simulink library "fmPlaneAttiIndi_lib"  (R2018b)
settings: Solver=VariableStepAuto  StartTime=0.0  StopTime=10.0  RelTol=1e-3
undefined symbols (not defined in the file or in its folder): DiscIntNeverNeededParam, fm_atti
libraries: filters_lib x3, ca_lib x1, sensors_lib x1, $bdroot x1
settings Model: Creator=Ybeyer  LastModifiedBy=yannic
settings SFSimCC: SimUseLocalCustomCode=off
settings RTWCC: RTWUseLocalCustomCode=off
settings CodeAppCC: StateflowObjectComments=on

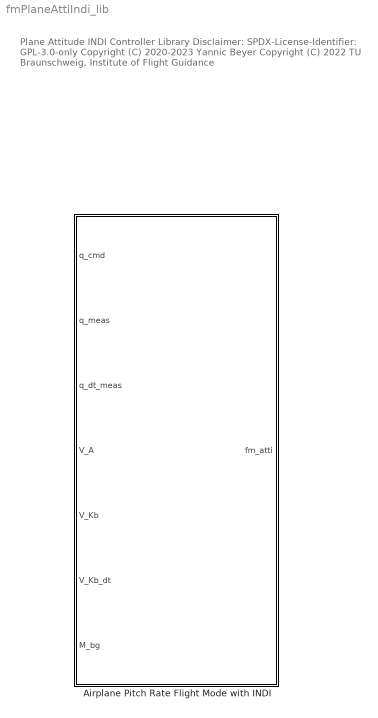
== system fmPlaneAttiIndi_lib ==
  note: Plane Attitude INDI Controller Library
      |
      | Disclaimer:
      | SPDX-License-Identifier: GPL-3.0-only
      |
      | Copyright (C) 2020-2023 Yannic Beyer
      | Copyright (C) 2022 TU Braunschweig, Institute of Flight Guidance
  Airplane Pitch Rate Flight Mode with INDI : Subsystem  mask{fm=fm_atti}
      mask prompts: fm "Multicopter Attitude Flight Mode (INDI) struct"
      mask DialogControl DescGroupVar Prompt: Multicopter Attitude Flight Mode with INDI and reduced attitude control
      mask DialogControl DescTextVar Prompt: Controller is basically implemented according to [1]
      mask DialogControl Control2 Prompt: [1] Sun, S., Baert, M., Van Schijndel, B. S., & De Visser, C. (2020, May). Upset Recovery Control for Quadrotors Subjected to a Complete Rotor Failure from Large Initial Disturbances. In 2020 IEEE International Conference on Robotics and Automation (ICRA) (pp. 4273-4279). IEEE.
      mask DialogControl Control3 Prompt: To initialize an attitude flight mode parameters struct see fmCopterAttiIndiLoadParams

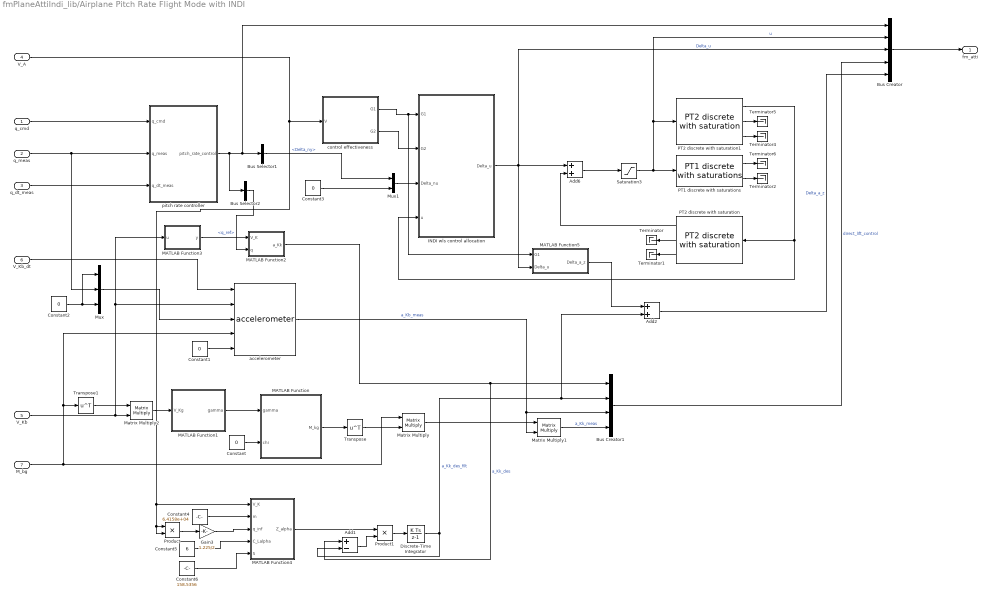
== system fmPlaneAttiIndi_lib/Airplane Pitch Rate Flight Mode with INDI ==
  q_cmd : Inport  SampleTime=fm.sample_time
  q_meas : Inport  Port=2  SampleTime=fm.sample_time
  q_dt_meas : Inport  Port=3  SampleTime=fm.sample_time
  V_A : Inport  Port=4  SampleTime=fm.sample_time
  V_Kb : Inport  Port=5  SampleTime=fm.sample_time
  V_Kb_dt : Inport  Port=6  SampleTime=fm.sample_time
  M_bg : Inport  Port=7  SampleTime=fm.sample_time
  Add1 : Sum  Inputs=+-
  Add2 : Sum
  Add6 : Sum
  Bus Creator : BusCreator  Inputs=5
  Bus Creator1 : BusCreator  Inputs=4
  Bus Selector1 : BusSelector  OutputSignals=pseudo_control.Delta_ny
  Bus Selector2 : BusSelector  OutputSignals=reference.q_ref
  Constant : Constant  Value=0
  Constant1 : Constant  Value=0  VectorParams1D=off
  Constant2 : Constant  Value=0
  Constant3 : Constant  Value=0
  Constant4 : Constant  Value=6.4158e+04
  Constant5 : Constant  Value=6
  Constant6 : Constant  Value=158.5356
  Discrete-Time Integrator : DiscreteIntegrator  SampleTime=-1  ICPrevOutput=DiscIntNeverNeededParam  ICPrevScaledInput=DiscIntNeverNeededParam
  Gain3 : Gain  Gain=1.225/2
  INDI wls control allocation : Subsystem  mask{ca=fm.ca, is_Delta_W_v_check=off, is_W_check=off, is_iter_check=off}
      mask prompts: ca "control allocation parameters struct"; is_Delta_W_v_check "enable online adjustment of diag W_v"; is_W_check "enable output "optimal active set" W"; is_iter_check "enable output "number of iterations" iter"
      mask init:
      | caIndiWlsHlcBlockInit(is_Delta_W_v_check,is_W_check,is_iter_check)
      mask DialogControl DescGroupVar Prompt: INDI high level control allocation
      mask DialogControl DescTextVar Prompt: It wraps the INDI control allocation block and adds some high level usability features.
      mask DialogControl Control2 Prompt: This block makes manual throttle control possible. Moreover, it not only considers the control effectiveness G1 but also the effectiveness of the control input derivative G2 [1].
      mask DialogControl Control3 Prompt: [1] Smeur, E. J., Chu, Q., & de Croon, G. C. (2016). Adaptive incremental nonlinear dynamic inversion for attitude control of micro air vehicles. Journal of Guidance, Control, and Dynamics, 39(3), 450-461.
      mask DialogControl Control4 Prompt: To load a control allocation parameters struct, see controlAllocationWlsLoadParams
  MATLAB Function : MATLAB Function  TreatAsAtomicUnit=on
  MATLAB Function1 : MATLAB Function  TreatAsAtomicUnit=on
  MATLAB Function2 : MATLAB Function  TreatAsAtomicUnit=on
  MATLAB Function3 : MATLAB Function  TreatAsAtomicUnit=on
  MATLAB Function4 : MATLAB Function  TreatAsAtomicUnit=on
  MATLAB Function5 : MATLAB Function  TreatAsAtomicUnit=on
  Matrix Multiply : Product  Multiplication=Matrix(*)
  Matrix Multiply1 : Product  Multiplication=Matrix(*)
  Matrix Multiply2 : Product  Multiplication=Matrix(*)
  Mux : Mux  Inputs=3
  Mux1 : Mux  Inputs=2
  PT1 discrete with saturations : filters_lib/PT1 discrete with saturations  T=fm.motor_time_constant  x_max=inf  x_min=-inf  x_dt_max=inf  x_dt_min=-inf  x_init=0
      settings: SourceProductName=LADAC
  PT2 discrete with saturation : filters_lib/PT2 discrete with saturation  param_src=internal  omega=fm.sens_filt.omega  d=fm.sens_filt.D  x_dt2_max=inf  x_dt2_min=-inf  x_dt_max=inf  x_dt_min=-inf  x_max=inf  x_min=-inf  y_0_src=internal  x_init=0  y_dt_0_src=internal  x_dt_init=0  is_y_dt_checked=on  is_y_dt2_checked=on
      settings: SourceProductName=LADAC
  PT2 discrete with saturation1 : filters_lib/PT2 discrete with saturation  param_src=internal  omega=fm.servo.omega  d=fm.servo.D  x_dt2_max=inf  x_dt2_min=-inf  x_dt_max=inf  x_dt_min=-inf  x_max=inf  x_min=-inf  y_0_src=internal  x_init=0  y_dt_0_src=internal  x_dt_init=0  is_y_dt_checked=on  is_y_dt2_checked=on
      settings: SourceProductName=LADAC
  Product : Product
  Product1 : Product
  Saturation3 : Saturate  UpperLimit=fm.ca.u_max  LowerLimit=fm.ca.u_min
  Terminator{,1..2,4..6} (6 alike) : Terminator
  Transpose : Math  Operator=transpose  SaturateOnIntegerOverflow=on
  Transpose1 : Math  Operator=transpose  SaturateOnIntegerOverflow=on
  accelerometer : sensors_lib/accelerometer  SystemSampleTime=-1
      settings: SourceProductName=LADAC
  control effectiveness : Subsystem
  pitch rate controller : Subsystem
  fm_atti : Outport  SampleTime=fm.sample_time
  wires:
  PT1 discrete with saturations/1 -> Terminator6/1
  PT2 discrete with saturation1/2 -> Terminator5/1
  PT2 discrete with saturation1/3 -> Terminator4/1
  PT2 discrete with saturation/1 -> Add6/2
  Bus Creator/1 -> fm_atti/1
  PT1 discrete with saturations/2 -> Terminator2/1
  PT2 discrete with saturation/3 -> Terminator1/1
  PT2 discrete with saturation/2 -> Terminator/1
  INDI wls control allocation/1(Delta_u) -> MATLAB Function5/2(Delta_u), Bus Creator/3, Add6/1  "Delta_u"
  control effectiveness/1(G1) -> MATLAB Function5/1(G1), INDI wls control allocation/1(G1)
  Add6/1 -> Saturation3/1
  control effectiveness/2(G2) -> INDI wls control allocation/2(G2)
  PT2 discrete with saturation1/1 -> INDI wls control allocation/4(u), PT2 discrete with saturation/1
  Bus Selector1/1 -> Mux1/1  "<Delta_ny>"
  Saturation3/1 -> Bus Creator/2, PT2 discrete with saturation1/1, PT1 discrete with saturations/1  "u"
  q_cmd/1 -> pitch rate controller/1(q_cmd)
  q_meas/1 -> Mux/2, pitch rate controller/2(q_meas)
  q_dt_meas/1 -> pitch rate controller/3(q_dt_meas)
  pitch rate controller/1(pitch_rate_control) -> Bus Selector2/1, Bus Creator/1, Bus Selector1/1
  V_A/1 -> Product/2, Product/1, MATLAB Function4/1(V_K), control effectiveness/1(V)
  V_Kb_dt/1 -> accelerometer/1
  MATLAB Function1/1(gamma) -> MATLAB Function/1(gamma)
  Constant/1 -> MATLAB Function/2(chi)
  M_bg/1 -> Matrix Multiply/1, accelerometer/4, Transpose1/1
  Constant1/1 -> accelerometer/5
  MATLAB Function/1(M_kg) -> Transpose/1
  Transpose/1 -> Matrix Multiply/2
  Matrix Multiply/1 -> Matrix Multiply1/1
  accelerometer/1 -> Matrix Multiply1/2, Bus Creator1/3  "a_Kb_meas"
  V_Kb/1 -> MATLAB Function3/1(u), accelerometer/2, Matrix Multiply2/2
  Constant2/1 -> Mux/1, Mux/3
  Mux/1 -> accelerometer/3
  Matrix Multiply1/1 -> Bus Creator1/4  "a_Kk_meas"
  Bus Creator1/1 -> Bus Creator/4  "direct_lift_control"
  MATLAB Function3/1(y) -> MATLAB Function2/1(V_K)
  MATLAB Function2/1(a_Kk) -> Add1/1, Bus Creator1/1  "a_Kk_des"
  Matrix Multiply2/1 -> MATLAB Function1/1(V_Kg)
  Transpose1/1 -> Matrix Multiply2/1
  Bus Selector2/1 -> MATLAB Function2/2(q)  "<q_ref>"
  Mux1/1 -> INDI wls control allocation/3(Delta_nu)
  Constant3/1 -> Mux1/2
  Constant4/1 -> MATLAB Function4/2(m)
  Product/1 -> Gain3/1
  Gain3/1 -> MATLAB Function4/3(q_inf)
  Constant5/1 -> MATLAB Function4/4(C_Lalpha)
  Constant6/1 -> MATLAB Function4/5(S)
  MATLAB Function4/1(Z_alpha) -> Product1/1
  Add1/1 -> Product1/2
  Product1/1 -> Discrete-Time Integrator/1
  Discrete-Time Integrator/1 -> Add2/2, Bus Creator1/2, Add1/2  "a_Kk_des_filt"
  MATLAB Function5/1(Delta_a_z) -> Add2/1
  Add2/1 -> Bus Creator/5  "Delta_a_z"

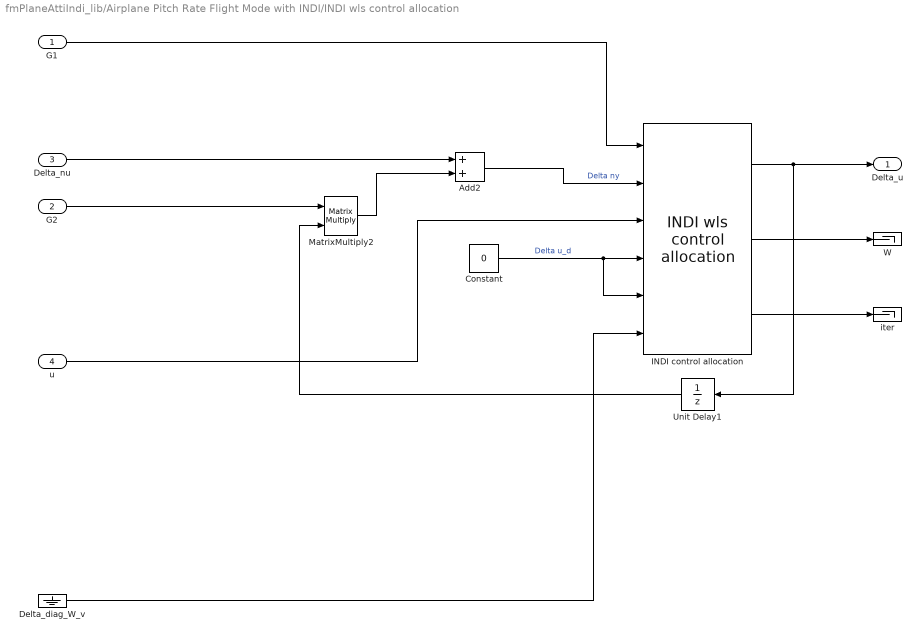
== system fmPlaneAttiIndi_lib/Airplane Pitch Rate Flight Mode with INDI/INDI wls control allocation ==
  G1 : Inport
  G2 : Inport  Port=2
  Delta_nu : Inport  Port=3
  u : Inport  Port=4
  Add2 : Sum
  Constant : Constant  Value=0
  Delta_diag_W_v : Ground
  INDI control allocation : ca_lib/INDI wls control allocation  ca=ca  is_Delta_u_d_checked=on  is_Delta_gamma_checked=on  is_Delta_W_v_checked=on  is_W_checked=on  is_iter_checked=on
      settings: SourceProductName=LADAC
  MatrixMultiply2 : Product  Multiplication=Matrix(*)
  Unit Delay1 : UnitDelay  SampleTime=-1
  W : Terminator
  iter : Terminator
  Delta_u : Outport
  wires:
  INDI control allocation/2 -> W/1
  INDI control allocation/3 -> iter/1
  Delta_diag_W_v/1 -> INDI control allocation/6
  Constant/1 -> INDI control allocation/5, INDI control allocation/4  "Delta u_d"
  Unit Delay1/1 -> MatrixMultiply2/2
  Delta_nu/1 -> Add2/1
  INDI control allocation/1 -> Delta_u/1, Unit Delay1/1
  u/1 -> INDI control allocation/3
  Add2/1 -> INDI control allocation/2  "Delta ny"
  G1/1 -> INDI control allocation/1
  MatrixMultiply2/1 -> Add2/2
  G2/1 -> MatrixMultiply2/1

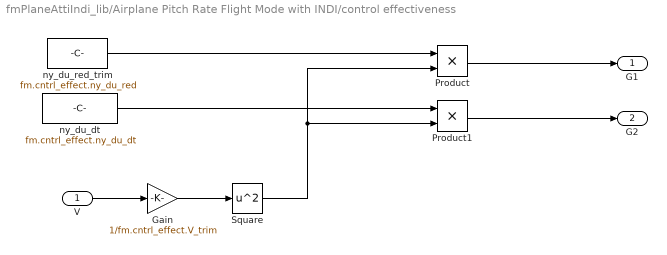
== system fmPlaneAttiIndi_lib/Airplane Pitch Rate Flight Mode with INDI/control effectiveness ==
  V : Inport
  Gain : Gain  Gain=1/fm.cntrl_effect.V_trim
  Product : Product
  Product1 : Product
  Square : Math  Operator=square  SaturateOnIntegerOverflow=on
  ny_du_dt : Constant  Value=fm.cntrl_effect.ny_du_dt
  ny_du_red_trim : Constant  Value=fm.cntrl_effect.ny_du_red
  G1 : Outport
  G2 : Outport  Port=2
  wires:
  Product1/1 -> G2/1
  Square/1 -> Product/2, Product1/2
  Product/1 -> G1/1
  Gain/1 -> Square/1
  V/1 -> Gain/1
  ny_du_red_trim/1 -> Product/1
  ny_du_dt/1 -> Product1/1

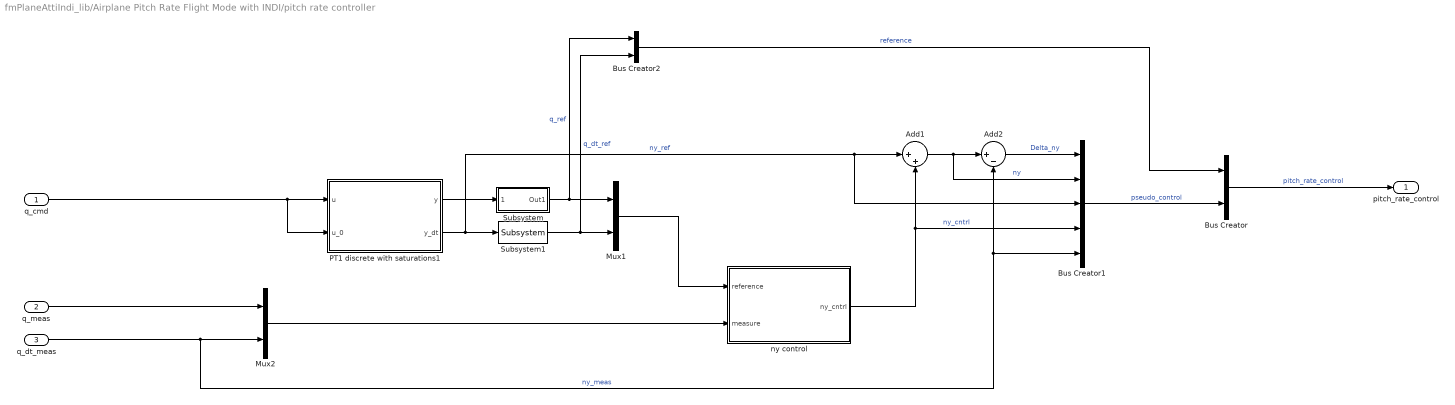
== system fmPlaneAttiIndi_lib/Airplane Pitch Rate Flight Mode with INDI/pitch rate controller ==
  q_cmd : Inport
  q_meas : Inport  Port=2
  q_dt_meas : Inport  Port=3
  Add1 : Sum  Inputs=|++
  Add2 : Sum  Inputs=|+-
  Bus Creator : BusCreator  Inputs=2
  Bus Creator1 : BusCreator  Inputs=5
  Bus Creator2 : BusCreator  Inputs=2
  Mux1 : Mux  Inputs=2
  Mux2 : Mux  Inputs=2
  PT1 discrete with saturations1 : Subsystem  mask{T=1/fm.atc.rm.leanfreq, x_max=inf, x_min=-inf, x_dt_max=inf, x_dt_min=-inf, x_init=0}
      mask prompts: T "Time constant"; x_max "Maximum output"; x_min "Minimum output"; x_dt_max "Maximum output rate"; x_dt_min "Minimum output rate"; x_init "Initial output"
  Subsystem : Subsystem
  Subsystem1 : $bdroot/Airplane Pitch Rate Flight Mode with INDI/pitch rate controller/Subsystem  SystemSampleTime=-1
  ny control : Subsystem
  pitch_rate_control : Outport
  wires:
  Mux1/1 -> ny control/1(reference)
  Add1/1 -> Add2/1, Bus Creator1/2  "ny"
  Bus Creator1/1 -> Bus Creator/2  "pseudo_control"
  PT1 discrete with saturations1/1(y) -> Subsystem/1(<x_ref>)
  Bus Creator/1 -> pitch_rate_control/1  "pitch_rate_control"
  Add2/1 -> Bus Creator1/1  "Delta_ny"
  PT1 discrete with saturations1/2(y_dt) -> Subsystem1/1, Bus Creator1/3, Add1/1  "ny_ref"
  Subsystem/1(Out1) -> Bus Creator2/1, Mux1/1  "q_ref"
  q_cmd/1 -> PT1 discrete with saturations1/2("u_0 "), PT1 discrete with saturations1/1(u)
  Subsystem1/1 -> Bus Creator2/2, Mux1/2  "q_dt_ref"
  q_meas/1 -> Mux2/1
  q_dt_meas/1 -> Add2/2, Bus Creator1/5, Mux2/2  "ny_meas"
  ny control/1(ny_cntrl) -> Bus Creator1/4, Add1/2  "ny_cntrl"
  Mux2/1 -> ny control/2(measure)
  Bus Creator2/1 -> Bus Creator/1  "reference"

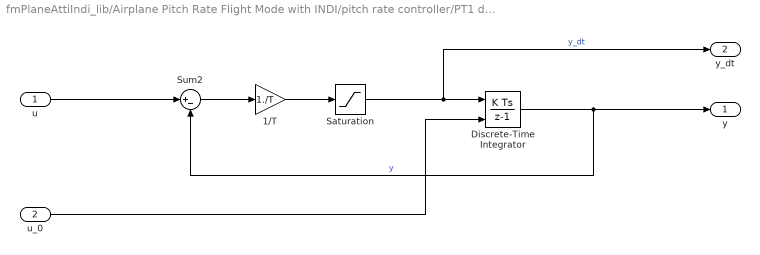
== system fmPlaneAttiIndi_lib/Airplane Pitch Rate Flight Mode with INDI/pitch rate controller/PT1 discrete with saturations1 ==
  u : Inport
  "u_0 " : Inport  Port=2
  1/T : Gain  Gain=1./T
  Discrete-Time Integrator : DiscreteIntegrator  InitialConditionSource=external  InitialCondition=x_init  SampleTime=-1  LimitOutput=on  UpperSaturationLimit=x_max  LowerSaturationLimit=x_min  ICPrevOutput=DiscIntNeverNeededParam  ICPrevScaledInput=DiscIntNeverNeededParam
  Saturation : Saturate  UpperLimit=x_dt_max  LowerLimit=x_dt_min
  Sum2 : Sum  Inputs=|+-
  y : Outport
  y_dt : Outport  Port=2
  wires:
  Saturation/1 -> Discrete-Time Integrator/1, y_dt/1  "y_dt"
  Discrete-Time Integrator/1 -> y/1, Sum2/2  "y"
  Sum2/1 -> 1/T/1
  u/1 -> Sum2/1
  1/T/1 -> Saturation/1
  "u_0 "/1 -> Discrete-Time Integrator/2

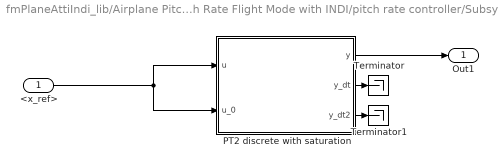
== system fmPlaneAttiIndi_lib/Airplane Pitch Rate Flight Mode with INDI/pitch rate controller/Subsystem ==
  <x_ref> : Inport
  PT2 discrete with saturation : Subsystem  mask{omega=2./(2/fm.sens_filt.omega + 2/fm.servo.omega), d=1, x_dt2_max=inf, x_dt2_min=-inf, x_dt_max=inf, x_dt_min=-inf, x_max=inf, x_min=-inf, x_init=0, x_dt_init=0}
      mask prompts: omega "Natural frequency"; d "Damping ratio"; x_dt2_max "Maximum acceleration"; x_dt2_min "Minimum acceleration"; x_dt_max "Maximum rate"; x_dt_min "Minimum rate"; x_max "Maximum position"; x_min "Minimum position"; x_init "Initial position"; x_dt_init "Initial rate"
  Terminator : Terminator
  Terminator1 : Terminator
  Out1 : Outport
  wires:
  <x_ref>/1 -> PT2 discrete with saturation/1(u), PT2 discrete with saturation/2(u_0)
  PT2 discrete with saturation/1(y) -> Out1/1
  PT2 discrete with saturation/3(y_dt2) -> Terminator1/1
  PT2 discrete with saturation/2(y_dt) -> Terminator/1

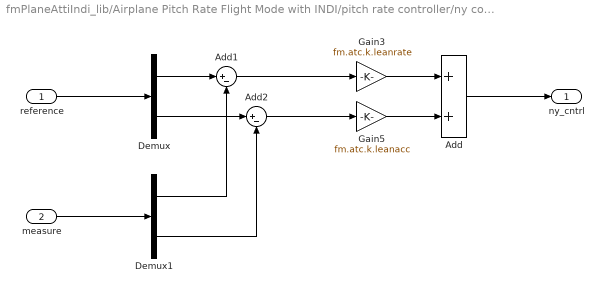
== system fmPlaneAttiIndi_lib/Airplane Pitch Rate Flight Mode with INDI/pitch rate controller/ny control ==
  reference : Inport
  measure : Inport  Port=2
  Add : Sum  Inputs=2
  Add1 : Sum  Inputs=|+-
  Add2 : Sum  Inputs=|+-
  Demux : Demux  Outputs=2
  Demux1 : Demux  Outputs=2
  Gain3 : Gain  Gain=fm.atc.k.leanrate
  Gain5 : Gain  Gain=fm.atc.k.leanacc
  ny_cntrl : Outport
  wires:
  Add/1 -> ny_cntrl/1
  Gain3/1 -> Add/1
  Gain5/1 -> Add/2
  Demux/2 -> Add2/1
  Demux/1 -> Add1/1
  reference/1 -> Demux/1
  measure/1 -> Demux1/1
  Add1/1 -> Gain3/1
  Add2/1 -> Gain5/1
  Demux1/1 -> Add1/2
  Demux1/2 -> Add2/2

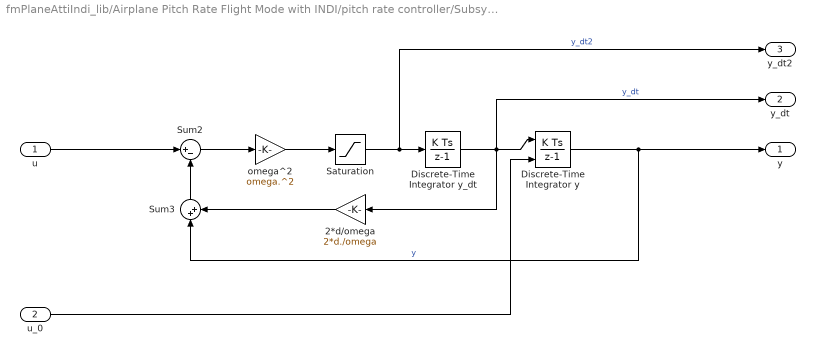
== system fmPlaneAttiIndi_lib/Airplane Pitch Rate Flight Mode with INDI/pitch rate controller/Subsystem/PT2 discrete with saturation ==
  u : Inport
  u_0 : Inport  Port=2
  2*d/omega : Gain  Gain=2*d./omega
  Discrete-Time Integrator y : DiscreteIntegrator  InitialConditionSource=external  InitialCondition=x_init  SampleTime=-1  OutDataTypeStr=Inherit: Inherit via back propagation  LimitOutput=on  UpperSaturationLimit=x_max  LowerSaturationLimit=x_min  ICPrevOutput=DiscIntNeverNeededParam  ICPrevScaledInput=DiscIntNeverNeededParam
  Discrete-Time Integrator y_dt : DiscreteIntegrator  InitialCondition=x_dt_init  SampleTime=-1  OutDataTypeStr=Inherit: Inherit via back propagation  LimitOutput=on  UpperSaturationLimit=x_dt_max  LowerSaturationLimit=x_dt_min  ICPrevOutput=DiscIntNeverNeededParam  ICPrevScaledInput=DiscIntNeverNeededParam
  Saturation : Saturate  UpperLimit=x_dt2_max  LowerLimit=x_dt2_min
  Sum2 : Sum  Inputs=|+-
  Sum3 : Sum  Inputs=|++
  omega^2 : Gain  Gain=omega.^2
  y : Outport
  y_dt : Outport  Port=2
  y_dt2 : Outport  Port=3
  wires:
  u_0/1 -> Discrete-Time Integrator y/2
  Discrete-Time Integrator y_dt/1 -> Discrete-Time Integrator y/1, y_dt/1, 2*d/omega/1  "y_dt"
  Discrete-Time Integrator y/1 -> y/1, Sum3/1  "y"
  Sum2/1 -> omega^2/1
  2*d/omega/1 -> Sum3/2
  u/1 -> Sum2/1
  Sum3/1 -> Sum2/2
  omega^2/1 -> Saturation/1
  Saturation/1 -> Discrete-Time Integrator y_dt/1, y_dt2/1  "y_dt2"

== matlab function fmPlaneAttiIndi_lib/Airplane Pitch Rate Flight Mode with INDI/MATLAB Function ==
  data: gamma input; M_kg output; chi input
function M_kg = dcmKgFromAngles(gamma,chi)
M_kg = dcmKgFromAngles(gamma,chi);
end

== matlab function fmPlaneAttiIndi_lib/Airplane Pitch Rate Flight Mode with INDI/MATLAB Function1 ==
  data: V_Kg input; gamma output
function gamma = flightPathAngle( V_Kg )
gamma = flightPathAngle( V_Kg );
end

== matlab function fmPlaneAttiIndi_lib/Airplane Pitch Rate Flight Mode with INDI/MATLAB Function2 ==
  data: V_K input; a_Kk output; q input
function a_Kk = fcn(V_K,q)
V_Kk = [V_K;0;0];
Omega_Kk = [0;q;0];
a_Kk = cross(Omega_Kk,V_Kk);
end

== matlab function fmPlaneAttiIndi_lib/Airplane Pitch Rate Flight Mode with INDI/MATLAB Function3 ==
  data: u input; y output
function y = fcn(u)
y=norm(u,2);
end

== matlab function fmPlaneAttiIndi_lib/Airplane Pitch Rate Flight Mode with INDI/MATLAB Function4 ==
  data: V_K input; Z_alpha output; m input; q_inf input; C_Lalpha input; S input
function Z_alpha = fcn(V_K,m,q_inf,C_Lalpha,S)

Z_alpha = 1/V_K*(1/m*q_inf*C_Lalpha*S);

end

== matlab function fmPlaneAttiIndi_lib/Airplane Pitch Rate Flight Mode with INDI/MATLAB Function5 ==
  data: G1 input; Delta_a_z output; Delta_u input
function Delta_a_z = fcn(G1, Delta_u)

% expected vertical acceleration due to elevator deflection
Delta_a_z = G1(2,3)*Delta_u(3);

end
